simulink model "Steer_Components"  (R2026b)
settings: Solver=VariableStepAuto
undefined symbols (not defined in the file): column_joints, qOffset, X, Y, Z
libraries: sm_lib x4
settings Model: Creator=smiller  LastModifiedBy=smiller

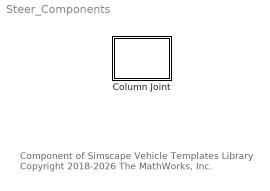
== system Steer_Components ==
  note: Component of Simscape Vehicle Templates Library
      | Copyright 2018-2026 The MathWorks, Inc.
  Column Joint : Subsystem  Variant=on  VariantControlMode=label  VariantControl=Choice  LabelModeActiveChoice=CV  mask{VariantLabel=column_joints, qOffset=qOffset}
      mask prompts: VariantLabel "Variant Label"; qOffset "Axis Rotation Offset (deg)"
      mask init:
      | curblk = gcb;
      | 
      | % Set variant for this block 
      | set_param(curblk,'LabelModeActiveChoice',VariantLabel);

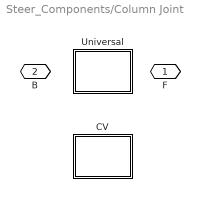
== system Steer_Components/Column Joint ==
  CV : Subsystem  VariantControl=CV
      mask Display: image('sm_car_variant_constant_velocity.png')
  Universal : Subsystem  VariantControl=Universal  mask{qOffset=qOffset}
      mask prompts: qOffset "Axis Rotation Offset (deg)"
      mask TypeOptions qOffset:
      | Transform
      | Orient Axes B/RotationAngle | Transform
      | Orient Axes F/RotationAngle
      mask Display: image('sm_car_variant_universal.png')
  F : PMIOPort  Side=Right
  B : PMIOPort  Port=2  Side=Left

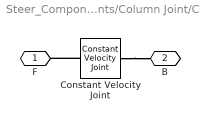
== system Steer_Components/Column Joint/CV ==
  Constant Velocity Joint : sm_lib/Joints/Constant Velocity Joint  JointMode=Normal  CompositeWrenchDir=FollowerOnBase  CompositeWrenchFrame=BaseFrame  SenseConstraintForce=off  SenseConstraintTorque=off  SenseTotalForce=off  SenseTotalTorque=off  InternalState=RotationSequence  PositionTargetSpecify=off  PositionTargetPriority=High  PositionTargetSpecificationMethod=BendAngleOnly  PositionTargetBendAngleValue=45  PositionTargetBendAngleValueUnits=deg  PositionTargetAzimuthValue=0.0  PositionTargetAzimuthValueUnits=deg  VelocityTargetSpecify=off  VelocityTargetPriority=High  VelocityTargetSpecificationMethod=BendAngleOnly  VelocityTargetBendAngleValue=0.0  VelocityTargetBendAngleValueUnits=deg/s  VelocityTargetAzimuthValue=0.0  VelocityTargetAzimuthValueUnits=deg/s  SenseBendAnglePosition=off  SenseBendAngleVelocity=off  SenseBendAngleAcceleration=off  SenseAzimuthPosition=off  SenseAzimuthVelocity=off  SenseAzimuthAcceleration=off
  F : PMIOPort  Side=Right
  B : PMIOPort  Port=2  Side=Left
  connections:
  Constant Velocity Joint/LConn1 -- B/RConn1
  Constant Velocity Joint/RConn1 -- F/RConn1

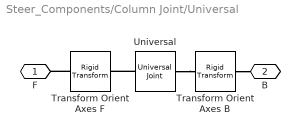
== system Steer_Components/Column Joint/Universal ==
  Transform Orient Axes B : sm_lib/Frames and Transforms/Rigid Transform  RotationMethod=StandardAxis  FollAlignAxisA=+X  BaseAlignAxisA=+Y  FollAlignAxisB=+Y  BaseAlignAxisB=+Z  RotationStandardAxis=+Z  RotationAngle=qOffset  RotationAngleUnits=deg  RotationArbitraryAxis=[0 0 1]  RotationSequenceAxes=FollowerAxes  RotationSequence=XYX  RotationSequenceAngles=[0 0 0]  RotationSequenceAnglesUnits=deg  RotationMatrix=[1 0 0; 0 1 0; 0 0 1]  Quaternion=[1 0 0 0]  TranslationMethod=None  TranslationCartesianOffset=[0 0 0]  TranslationCartesianOffsetUnits=m  TranslationStandardAxis=+Z  TranslationStandardOffset=0  TranslationStandardOffsetUnits=m  TranslationROffset=0  TranslationROffsetUnits=m  TranslationThetaOffset=0  TranslationThetaOffsetUnits=deg  TranslationZOffset=0  TranslationZOffsetUnits=m
  Transform Orient Axes F : sm_lib/Frames and Transforms/Rigid Transform  RotationMethod=StandardAxis  FollAlignAxisA=+X  BaseAlignAxisA=+Y  FollAlignAxisB=+Y  BaseAlignAxisB=+Z  RotationStandardAxis=+Z  RotationAngle=qOffset  RotationAngleUnits=deg  RotationArbitraryAxis=[0 0 1]  RotationSequenceAxes=FollowerAxes  RotationSequence=XYX  RotationSequenceAngles=[0 0 0]  RotationSequenceAnglesUnits=deg  RotationMatrix=[1 0 0; 0 1 0; 0 0 1]  Quaternion=[1 0 0 0]  TranslationMethod=None  TranslationCartesianOffset=[0 0 0]  TranslationCartesianOffsetUnits=m  TranslationStandardAxis=+Z  TranslationStandardOffset=0  TranslationStandardOffsetUnits=m  TranslationROffset=0  TranslationROffsetUnits=m  TranslationThetaOffset=0  TranslationThetaOffsetUnits=deg  TranslationZOffset=0  TranslationZOffsetUnits=m
  Universal : sm_lib/Joints/Universal Joint  JointMode=Normal  CompositeWrenchDir=FollowerOnBase  CompositeWrenchFrame=BaseFrame  SenseConstraintForce=off  SenseConstraintTorque=off  SenseTotalForce=off  SenseTotalTorque=off  RxPositionTargetSpecify=off  RxPositionTargetPriority=High  RxPositionTargetValue=0  RxPositionTargetValueUnits=deg  RxVelocityTargetSpecify=off  RxVelocityTargetPriority=High  RxVelocityTargetValue=0  RxVelocityTargetValueUnits=deg/s  RxEquilibriumPosition=0  RxEquilibriumPositionUnits=deg  RxSpringStiffness=0  RxSpringStiffnessUnits=N*m/deg  RxDampingCoefficient=0  RxDampingCoefficientUnits=N*m/(deg/s)  RxLowerLimitSpecify=off  RxLowerLimitBound=-90  RxLowerLimitBoundUnits=deg  RxLowerLimitStiffness=1e4  RxLowerLimitStiffnessUnits=N*m/deg  RxLowerLimitDamping=10  RxLowerLimitDampingUnits=N*m/(deg/s)  RxLowerLimitTransitionRegionWidth=0.1  RxLowerLimitTransitionRegionWidthUnits=deg  RxUpperLimitSpecify=off  RxUpperLimitBound=90  RxUpperLimitBoundUnits=deg  RxUpperLimitStiffness=1e4  RxUpperLimitStiffnessUnits=N*m/deg  RxUpperLimitDamping=10  RxUpperLimitDampingUnits=N*m/(deg/s)  RxUpperLimitTransitionRegionWidth=0.1  RxUpperLimitTransitionRegionWidthUnits=deg  RxTorqueActuationMode=NoTorque  RxMotionActuationMode=ComputedMotion  RxSensePosition=off  RxSenseVelocity=off  RxSenseAcceleration=off  RxSenseTorqueForce=off  RxSenseLowerLimitTorqueForce=off  RxSenseUpperLimitTorqueForce=off  RyPositionTargetSpecify=off  RyPositionTargetPriority=High  RyPositionTargetValue=0  RyPositionTargetValueUnits=deg  RyVelocityTargetSpecify=off  RyVelocityTargetPriority=High  RyVelocityTargetValue=0  RyVelocityTargetValueUnits=deg/s  RyEquilibriumPosition=0  RyEquilibriumPositionUnits=deg  RySpringStiffness=0  RySpringStiffnessUnits=N*m/deg  RyDampingCoefficient=0  RyDampingCoefficientUnits=N*m/(deg/s)  RyLowerLimitSpecify=off  RyLowerLimitBound=-90  RyLowerLimitBoundUnits=deg  RyLowerLimitStiffness=1e4  RyLowerLimitStiffnessUnits=N*m/deg  RyLowerLimitDamping=10  RyLowerLimitDampingUnits=N*m/(deg/s)  RyLowerLimitTransitionRegionWidth=0.1  RyLowerLimitTransitionRegionWidthUnits=deg  RyUpperLimitSpecify=off  RyUpperLimitBound=90  RyUpperLimitBoundUnits=deg  RyUpperLimitStiffness=1e4  RyUpperLimitStiffnessUnits=N*m/deg  RyUpperLimitDamping=10  RyUpperLimitDampingUnits=N*m/(deg/s)  RyUpperLimitTransitionRegionWidth=0.1  RyUpperLimitTransitionRegionWidthUnits=deg  RyTorqueActuationMode=NoTorque  RyMotionActuationMode=ComputedMotion  RySensePosition=off  RySenseVelocity=off  RySenseAcceleration=off  RySenseTorqueForce=off  RySenseLowerLimitTorqueForce=off  RySenseUpperLimitTorqueForce=off
  F : PMIOPort  Side=Right
  B : PMIOPort  Port=2  Side=Left
  connections:
  Universal/RConn1 -- Transform Orient Axes F/RConn1
  Transform Orient Axes B/LConn1 -- B/RConn1
  Transform Orient Axes F/LConn1 -- F/RConn1
  Universal/LConn1 -- Transform Orient Axes B/RConn1
